simulink model "Intelligent_Battery_MPC_R2025b"  (R2025b)
settings: Solver=VariableStepAuto  StartTime=0.0  StopTime=8000  RelTol=1e-3
InitFcn:
  | run(fullfile(fileparts(get_param(bdroot,'FileName')),'setup_mpc_controller.m'))
undefined symbols (not defined in the file or in its folder): Ion, Lithium
libraries: spsMosfetLib x2, spsBatteryLib x1, spsDCVoltageSourceLib x1, mpclib x1, slpidlib x1, spsPWMGeneratorDCDCLib x1, spsSeriesRLCBranchLib x1, spspowerguiLib x1
settings Model: Creator=parinita  LastModifiedBy=iamam

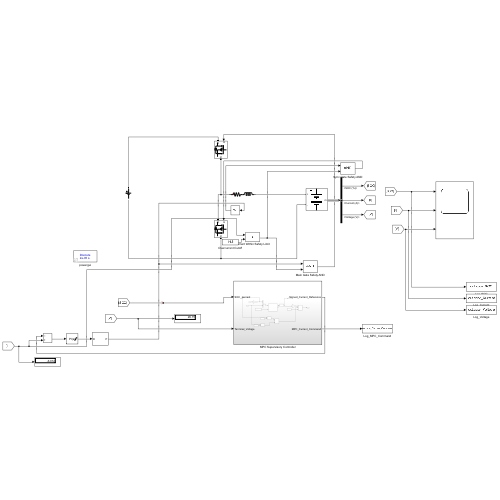
[thumbnail: Simulink's stored preview of the top-level diagram]
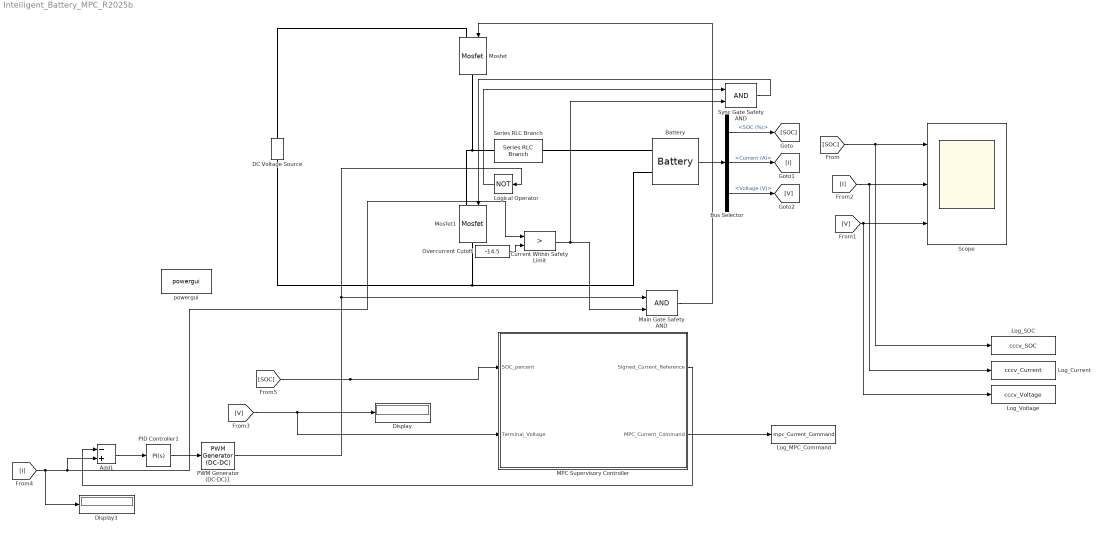
== system Intelligent_Battery_MPC_R2025b ==
  Add1 : Sum  Inputs=-+
  Battery : spsBatteryLib/Battery  BatType=Lithium-Ion  NomV=24  NomQ=20  SOC=70  Batt_Tr=1  PresetModel=on  MaxQ=20  MinV=18  FullV=27.9357  Dis_rate=8.6957  R=0.012  Normal_OP=18.087  expZone="[25.9293     0.982609]"
  Bus Selector : BusSelector  OutputSignals=SOC (%),Current (A),Voltage (V)
  Current Within Safety Limit : RelationalOperator  Operator=>  OutDataTypeStr=boolean  RndMeth=Simplest  InputSameDT=off
  DC Voltage Source : spsDCVoltageSourceLib/DC Voltage Source  Amplitude=36  Measurements=None
  Display : Display
  Display3 : Display
  Log_Current : ToWorkspace  VariableName=cccv_Current  SaveFormat=Timeseries  SampleTime=-1
      settings: MaxDataPoints=1e7
  Log_MPC_Command : ToWorkspace  VariableName=mpc_Current_Command  SaveFormat=Timeseries  SampleTime=-1
      settings: MaxDataPoints=1e7
  Log_SOC : ToWorkspace  VariableName=cccv_SOC  SaveFormat=Timeseries  SampleTime=-1
      settings: MaxDataPoints=1e7
  Log_Voltage : ToWorkspace  VariableName=cccv_Voltage  SaveFormat=Timeseries  SampleTime=-1
      settings: MaxDataPoints=1e7
  Logical Operator : Logic  Operator=NOT  AllPortsSameDT=off  OutDataTypeStr=boolean
  MPC Supervisory Controller : Subsystem
  Main Gate Safety AND : Logic  AllPortsSameDT=off  OutDataTypeStr=boolean
  Mosfet : spsMosfetLib/Mosfet  Ron=0.1  Lon=0  Rd=0.01  Vfd=0  IC=0  Rs=1e5  Cs=inf  Measurements=off
  Mosfet1 : spsMosfetLib/Mosfet  Ron=0.1  Lon=0  Rd=0.01  Vfd=0  IC=0  Rs=1e5  Cs=inf  Measurements=off
  Overcurrent Cutoff : Constant  Value=-14.5
  PID Controller1 : slpidlib/PID Controller  Controller=PI  Form=Parallel  TimeDomain=Continuous-time  UseExternalTs=off  SampleTime=-1  IntegratorMethod=Forward Euler  FilterMethod=Forward Euler  ControllerParametersSource=internal  P=0.01  I=2  UseKiTs=off  D=0  UseExternalDerivativeSource=off  N=100  UseFilter=on  TunerSelectOption=Transfer Function Based (PID Tuner App)  InitialConditionSource=internal  InitialConditionForIntegrator=0  InitialConditionForFilter=0  DifferentiatorICPrevScaledInput=0  ExternalReset=none  TrackingMode=off  Kt=1  LimitOutput=on  SatLimitsSource=internal  UpperSaturationLimit=1  LowerSaturationLimit=0  LinearizeAsGain=on  AntiWindupMode=back-calculation  Kb=1  LimitIntegrator=off  UpperIntegratorSaturationLimit=inf  LowerIntegratorSaturationLimit=-inf  POutMin=[]  POutMax=[]  IOutMin=[]  IOutMax=[]  DOutMin=[]  DOutMax=[]  NOutMin=[]  NOutMax=[]  SumOutMin=[]  SumOutMax=[]  SaturationOutMin=[]  SaturationOutMax=[]  PParamMin=[]  PParamMax=[]  IParamMin=[]  IParamMax=[]  DParamMin=[]  DParamMax=[]  NParamMin=[]  NParamMax=[]  KbParamMin=[]  KbParamMax=[]  KtParamMin=[]  KtParamMax=[]  KbOutMin=[]  KbOutMax=[]  KtOutMin=[]  KtOutMax=[]  IntegratorOutMin=[]  IntegratorOutMax=[]  FilterOutMin=[]  FilterOutMax=[]  SumI1OutMin=[]  SumI1OutMax=[]  SumI2OutMin=[]  SumI2OutMax=[]  SumI3OutMin=[]  SumI3OutMax=[]  SumI4OutMin=[]  SumI4OutMax=[]  SumDOutMin=[]  SumDOutMax=[]  DifferentiatorOutMin=[]  DifferentiatorOutMax=[]  FilterDiffOutCoefMin=[]  FilterDiffOutCoefMax=[]  ReciprocalOutMin=[]  ReciprocalOutMax=[]  SumDenOutMin=[]  SumDenOutMax=[]  SumNumOutMin=[]  SumNumOutMax=[]  DivideOutMin=[]  DivideOutMax=[]  UdiffTsProdOutMin=[]  UdiffTsProdOutMax=[]  NTsProdOutMin=[]  NTsProdOutMax=[]  UintegralTsProdOutMin=[]  UintegralTsProdOutMax=[]  UngainTsProdOutMin=[]  UngainTsProdOutMax=[]  ClampingZeroOutDataTypeStr=Inherit: Inherit via back propagation  ClampingZeroOutMin=[]  ClampingZeroOutMax=[]  FilterDenConstantOutDataTypeStr=Inherit: Inherit via back propagation  FilterDenConstantOutMin=[]  FilterDenConstantOutMax=[]  PCopyOutDataTypeStr=Inherit: Inherit via back propagation  PCopyOutMin=[]  PCopyOutMax=[]  NCopyOutDataTypeStr=Inherit: Inherit via back propagation  NCopyOutMin=[]  NCopyOutMax=[]  IntegratorContinuousStateAttributes=''  IntegratorStateMustResolveToSignalObject=off  IntegratorRTWStateStorageClass=Auto  FilterContinuousStateAttributes=''  FilterStateMustResolveToSignalObject=off  FilterRTWStateStorageClass=Auto  ParallelPVariant=InternalParameters  IdealPVariant=Disabled  IVariant=InternalParameters  DVariant=Disabled  IntegratorVariant=Continuous  SatVariant=Enabled  AWVariant=BackCalculation  PCopyVariant=Disabled  TRVariant=Disabled  FdbkBlocksVariant=Forward  IdealPFdbkVariant=Disabled  SatFdbkVariant=Disabled  DerivativeFilterVariant=Disabled  NVariant=Disabled  NCopyVariant=Disabled_SignalSpec  FilterICVariant=Disabled  IntegratorICVariant=InternalICs  ExternalResetVariant=Disabled  TRSumVariant=Passthrough  SumFdbkVariant=Disabled  SumVariant=Sum_PI  TsampFilterVariant=InternalTs  TsampNgainVariant=Passthrough  TsampIntegralVariant=Disabled_SignalSpec  ExternalSaturationOutDataTypeStr=Inherit: Same as second input  DerivativeSourceVariant=Disabled  PreIntVariant=InternalPreInt
  PWM Generator (DC-DC)1 : spsPWMGeneratorDCDCLib/PWM Generator (DC-DC)  Fsw=10e3  Ts=20e-6
  Scope : Scope  NumInputPorts=3
      settings: ActiveDisplayString=3  ActiveDisplayYMinimum=-2.1179170387001065  ActiveDisplayYMaximum=34.913242770607887
  Series RLC Branch : spsSeriesRLCBranchLib/Series RLC Branch  LConnTagsString=__new0  RConnTagsString=__new0  BranchType=RL  Resistance=0.05  Inductance=10e-3  SetiL0=off  InitialCurrent=0  Capacitance=1e-6  Setx0=off  InitialVoltage=0  Measurements=None
  Sync Gate Safety AND : Logic  AllPortsSameDT=off  OutDataTypeStr=boolean
  powergui : spspowerguiLib/powergui  Priority=1  SimulationMode=Discrete  SampleTime=20e-6  frequency=60  Iterations=50  frequencyindice=0  Pbase=100e6  ErrMax=1e-4  UnitsV=kV  UnitsW=MW  buscounter=0  FunctionMessages=off  echomessages=off  EnableUseOfTLC=off  CurrentSourceSwitches=off  DisableSnubberDevices=off  DisableRonSwitches=off  DisableVfSwitches=off  DisplayEquations=off  AutomaticDiscreteSolvers=off  SolverType=Tustin/Backward Euler (TBE)  Interpol=off  ExternalGateDelay=off  methode=off  Ts=100  x0status=blocks  SPID=on  SwTol=0  HookPort=off  NonlinearTolerance=1e-4  nMaxIteration=100  ContinueOnMaxIteration=off  RestoreLinks=warning  ResistiveCurrentMeasurement=off  Frange=[0:2:500]  Ylog=off  Xlog=on  ShowGrid=off  save=off  variable=ZData  structure=0  ZoomFFT=off  StartTime=0.0  cycles=1  DisplayStyle=1  fundamental=60  FreqAxis=off  MaxFrequency=1000  frequencyindicesteady=1  RmsSteady=1  display=off
  wires:
  [I] -> Current Within Safety Limit/1, Add1/2, Display3/1
  Bus Selector/2 -> [I]  "<Current (A)>"
  Bus Selector/1 -> [SOC]  "<SOC (%)>"
  Battery/1 -> Bus Selector/1
  Add1/1 -> PID Controller1/1
  Bus Selector/3 -> [V]  "<Voltage (V)>"
  [I] -> Scope/2, Log_Current/1
  [SOC] -> MPC Supervisory Controller/1(SOC_percent)
  [V] -> MPC Supervisory Controller/2(Terminal_Voltage), Display/1
  [SOC] -> Scope/1, Log_SOC/1
  [V] -> Scope/3, Log_Voltage/1
  PWM Generator (DC-DC)1/1 -> Logical Operator/1, Main Gate Safety AND/1
  Overcurrent Cutoff/1 -> Current Within Safety Limit/2
  Current Within Safety Limit/1 -> Main Gate Safety AND/2, Sync Gate Safety AND/2
  Logical Operator/1 -> Sync Gate Safety AND/1
  Main Gate Safety AND/1 -> Mosfet/1
  Sync Gate Safety AND/1 -> Mosfet1/1
  PID Controller1/1 -> PWM Generator (DC-DC)1/1
  MPC Supervisory Controller/1(Signed_Current_Reference) -> Add1/1
  MPC Supervisory Controller/2(MPC_Current_Command) -> Log_MPC_Command/1
  connections:
  Mosfet1/RConn1 -- Battery/LConn2 -- DC Voltage Source/LConn1
  Mosfet/RConn1 -- Series RLC Branch/LConn1 -- Mosfet1/LConn1
  DC Voltage Source/RConn1 -- Mosfet/LConn1
  Battery/LConn1 -- Series RLC Branch/RConn1

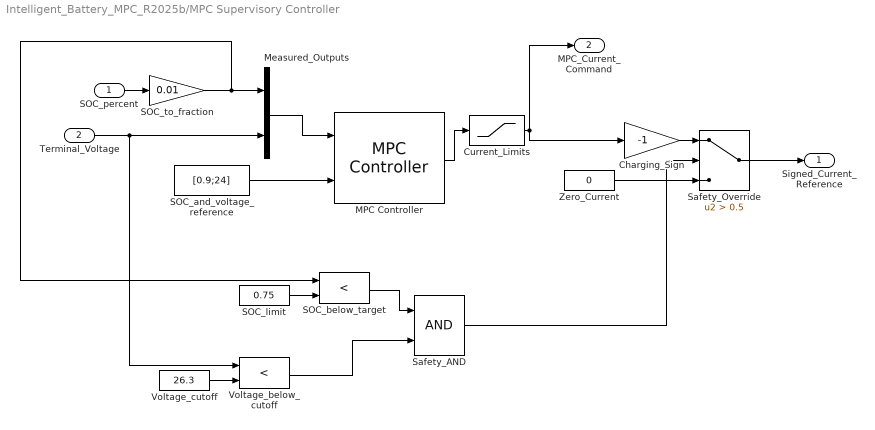
== system Intelligent_Battery_MPC_R2025b/MPC Supervisory Controller ==
  SOC_percent : Inport
  Terminal_Voltage : Inport  Port=2
  Charging_Sign : Gain  Gain=-1
  Current_Limits : Saturate  UpperLimit=13.5  LowerLimit=0
  MPC Controller : mpclib/MPC Controller  SCDEnableBlockLinearizationSpecification=on  mpcobj=batteryMPC  is_multiple=0  enable_value=0  return_u0=off  updateMPCinCallerWorkspace=on  md_inport=off  mv_inport=off  uref_inport=off  return_cost=off  return_mvseq=off  return_qpstatus=off  return_xseq=off  return_state=off  return_ovseq=off  state_inport=off  umin_inport=off  umax_inport=off  ymin_inport=off  ymax_inport=off  cc_inport=off  ywt_inport=off  uwt_inport=off  duwt_inport=off  rhoeps_inport=off  pm_inport=off  MaximumP=10  HorizonChoice=FixedHorizon  n_ts=1  n_p=30  n_mv=1  n_md=0  n_ud=0  n_mo=2  n_uo=0  BlockDataType=double  SampleTimeInherited=off  switch_inport=off
  Measured_Outputs : Mux  Inputs=2
  SOC_and_voltage_reference : Constant  Value=[0.9;24]
  SOC_below_target : RelationalOperator  Operator=<  OutDataTypeStr=boolean  RndMeth=Simplest  InputSameDT=off
  SOC_limit : Constant  Value=0.75
  SOC_to_fraction : Gain  Gain=0.01
  Safety_AND : Logic  AllPortsSameDT=off  OutDataTypeStr=boolean
  Safety_Override : Switch  Criteria=u2 > Threshold  Threshold=0.5  SaturateOnIntegerOverflow=off  InputSameDT=off
  Voltage_below_cutoff : RelationalOperator  Operator=<  OutDataTypeStr=boolean  RndMeth=Simplest  InputSameDT=off
  Voltage_cutoff : Constant  Value=26.3
  Zero_Current : Constant  Value=0
  Signed_Current_Reference : Outport
  MPC_Current_Command : Outport  Port=2
  wires:
  SOC_percent/1 -> SOC_to_fraction/1
  SOC_to_fraction/1 -> SOC_below_target/1, Measured_Outputs/1
  Terminal_Voltage/1 -> Voltage_below_cutoff/1, Measured_Outputs/2
  Measured_Outputs/1 -> MPC Controller/1
  SOC_and_voltage_reference/1 -> MPC Controller/2
  MPC Controller/1 -> Current_Limits/1
  Current_Limits/1 -> Charging_Sign/1, MPC_Current_Command/1
  Charging_Sign/1 -> Safety_Override/1
  Safety_AND/1 -> Safety_Override/2
  Zero_Current/1 -> Safety_Override/3
  Safety_Override/1 -> Signed_Current_Reference/1
  SOC_limit/1 -> SOC_below_target/2
  Voltage_cutoff/1 -> Voltage_below_cutoff/2
  SOC_below_target/1 -> Safety_AND/1
  Voltage_below_cutoff/1 -> Safety_AND/2
